simulink model "sim_config2a_trim"  (R2023b)
settings: Solver=ode4  StartTime=0.0  StopTime=60  FixedStep=0.01  RelTol=1e-3
undefined symbols (not defined in the file): aircraft, alt_ground, atmosphere, envir, g, pos_ref, wind
libraries: atmosphere_lib x1, flightgear_visualization_lib x1, syntrac_lib x1
settings Model: Creator=yannic  LastModifiedBy=yannic
settings DebuggingCC: InitInArrayFormatMsg=none

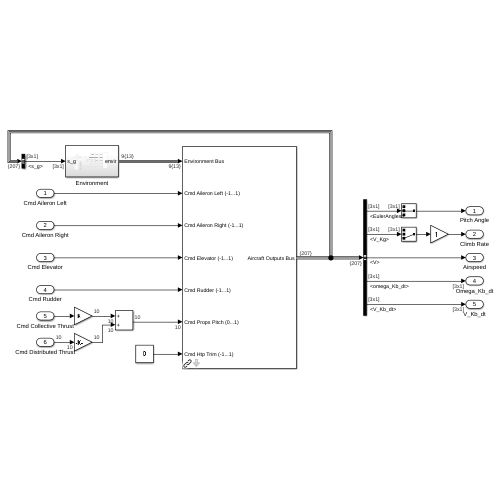
[thumbnail: Simulink's stored preview of the top-level diagram]
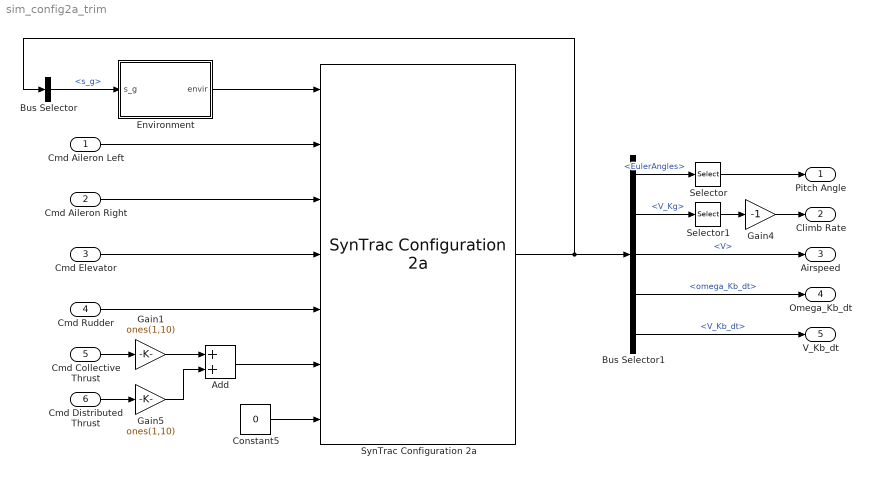
== system sim_config2a_trim ==
  Cmd Aileron Left : Inport
  Cmd Aileron Right : Inport  Port=2
  Cmd Elevator : Inport  Port=3
  Cmd Rudder : Inport  Port=4
  Cmd Collective Thrust : Inport  Port=5
  Cmd Distributed Thrust : Inport  Port=6  PortDimensions=length(aircraft.prop)
  Add : Sum
  Bus Selector : BusSelector  OutputSignals=rigidBodyBus.s_g
  Bus Selector1 : BusSelector  OutputSignals=rigidBodyBus.EulerAngles,rigidBodyBus.V_Kg,aeroBus.main.body.V,rigidBodyBus.omega_Kb_dt,rigidBodyBus.V_Kb_dt
  Constant5 : Constant  Value=0
  Environment : Subsystem
  Gain1 : Gain  Gain=ones(1,10)
  Gain4 : Gain  Gain=-1
  Gain5 : Gain  Gain=ones(1,10)
  Selector : Selector  InputPortWidth=3  IndexOptions=Index vector (dialog)  Indices=2  OutputSizes=1
  Selector1 : Selector  InputPortWidth=3  IndexOptions=Index vector (dialog)  Indices=3  OutputSizes=1
  SynTrac Configuration 2a : syntrac_lib/SynTrac Configuration 2a  aircraft=aircraft  ic=ic
  Pitch Angle : Outport
  Climb Rate : Outport  Port=2
  Airspeed : Outport  Port=3
  Omega_Kb_dt : Outport  Port=4
  V_Kb_dt : Outport  Port=5
  wires:
  Environment/1(envir) -> SynTrac Configuration 2a/1
  SynTrac Configuration 2a/1 -> Bus Selector1/1, Bus Selector/1
  Bus Selector/1 -> Environment/1(s_g)  "<s_g>"
  Cmd Aileron Right/1 -> SynTrac Configuration 2a/3
  Add/1 -> SynTrac Configuration 2a/6
  Constant5/1 -> SynTrac Configuration 2a/7
  Cmd Elevator/1 -> SynTrac Configuration 2a/4
  Cmd Rudder/1 -> SynTrac Configuration 2a/5
  Bus Selector1/1 -> Selector/1  "<EulerAngles>"
  Selector/1 -> Pitch Angle/1
  Bus Selector1/2 -> Selector1/1  "<V_Kg>"
  Selector1/1 -> Gain4/1
  Gain4/1 -> Climb Rate/1
  Bus Selector1/3 -> Airspeed/1  "<V>"
  Cmd Collective Thrust/1 -> Gain1/1
  Cmd Distributed Thrust/1 -> Gain5/1
  Bus Selector1/4 -> Omega_Kb_dt/1  "<omega_Kb_dt>"
  Bus Selector1/5 -> V_Kb_dt/1  "<V_Kb_dt>"
  Gain1/1 -> Add/1
  Gain5/1 -> Add/2
  Cmd Aileron Left/1 -> SynTrac Configuration 2a/2

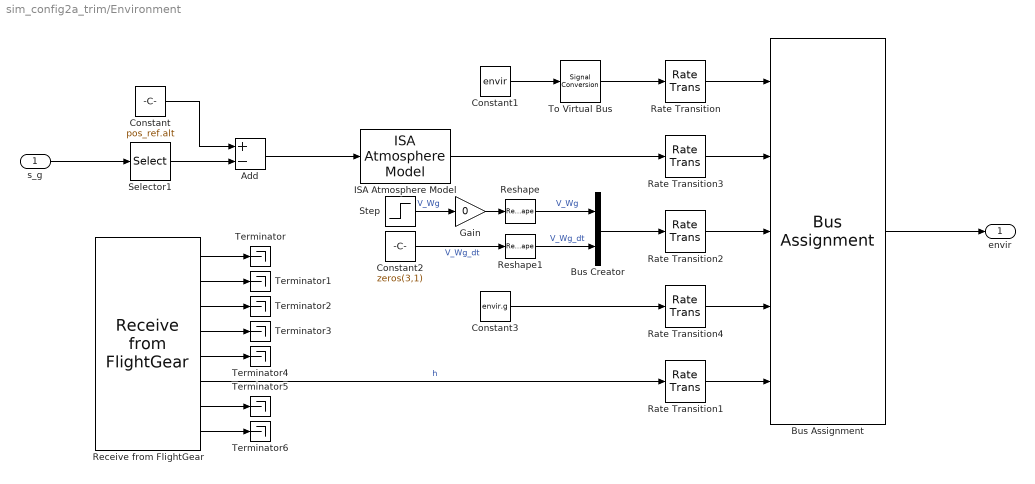
== system sim_config2a_trim/Environment ==
  s_g : Inport
  Add : Sum  Inputs=+-
  Bus Assignment : BusAssignment  AssignedSignals=atmosphere,wind,g,alt_ground
  Bus Creator : BusCreator  Inputs=2
  Constant : Constant  Value=pos_ref.alt
  Constant1 : Constant  Value=envir  OutDataTypeStr=Bus: envirBus
  Constant2 : Constant  Value=zeros(3,1)
  Constant3 : Constant  Value=envir.g
  Gain : Gain  Gain=0
  ISA Atmosphere Model : atmosphere_lib/ISA Atmosphere Model
      settings: SourceProductName=LADAC
  Rate Transition{,1..4} (5 alike) : RateTransition
  Receive from FlightGear : flightgear_visualization_lib/Receive from FlightGear  ip_address='127.0.0.1'  ip_port=5503  sample_time=1/20  blocking_time=0  is_aerocntrl=off  is_engine=off  is_fuel=off  is_land=off  is_avionics=off  is_envir=on
      settings: SourceProductName=LADAC
  Reshape : Reshape  OutputDimensionality=Column vector (2-D)
  Reshape1 : Reshape  OutputDimensionality=Column vector (2-D)
  Selector1 : Selector  InputPortWidth=3  IndexOptions=Index vector (dialog)  Indices=3  OutputSizes=1
  Step : Step  Time=3  After=[0;9;0]  SampleTime=0
  Terminator{,1..6} (7 alike) : Terminator
  To Virtual Bus : SignalConversion  ConversionOutput=Virtual bus  OverrideOpt=off
  envir : Outport  VectorParamsAs1DForOutWhenUnconnected=off
  wires:
  Rate Transition2/1 -> Bus Assignment/3
  Rate Transition3/1 -> Bus Assignment/2
  Bus Assignment/1 -> envir/1
  Rate Transition/1 -> Bus Assignment/1
  ISA Atmosphere Model/1 -> Rate Transition3/1
  Step/1 -> Gain/1  "V_Wg"
  Rate Transition1/1 -> Bus Assignment/5
  Constant1/1 -> To Virtual Bus/1
  s_g/1 -> Selector1/1
  Bus Creator/1 -> Rate Transition2/1
  Constant2/1 -> Reshape1/1  "V_Wg_dt"
  Rate Transition4/1 -> Bus Assignment/4
  Constant3/1 -> Rate Transition4/1
  Gain/1 -> Reshape/1
  Constant/1 -> Add/1
  Add/1 -> ISA Atmosphere Model/1
  Selector1/1 -> Add/2
  To Virtual Bus/1 -> Rate Transition/1
  Reshape/1 -> Bus Creator/1  "V_Wg"
  Reshape1/1 -> Bus Creator/2  "V_Wg_dt"
  Receive from FlightGear/3 -> Terminator2/1
  Receive from FlightGear/1 -> Terminator/1
  Receive from FlightGear/6 -> Rate Transition1/1  "h"
  Receive from FlightGear/2 -> Terminator1/1
  Receive from FlightGear/5 -> Terminator4/1
  Receive from FlightGear/7 -> Terminator5/1
  Receive from FlightGear/4 -> Terminator3/1
  Receive from FlightGear/8 -> Terminator6/1
